simulink model "Battery_16EV_Cascaded_ACBus"  (R2026a)
settings: Solver=ode23t  StopTime=2
PreLoadFcn:
  | load('battery_pack_parameters.mat')
values from neighbouring files (symbols this model uses):
  branchSOH = [0.8 0.85 0.9 0.95 0.82 0.87 0.92 0.97 0.78 0.88 0.93 1 ... (16 elements, 1x16)]    [battery_pack_parameters.mat]
  packs =     [battery_bms_parameters.mat]    (also in battery_pack_parameters.mat)
libraries: fl_lib x145, nesl_utility x128, ee_lib x80, simulink x17, batteryecm_lib x16
(part 3 of 16)

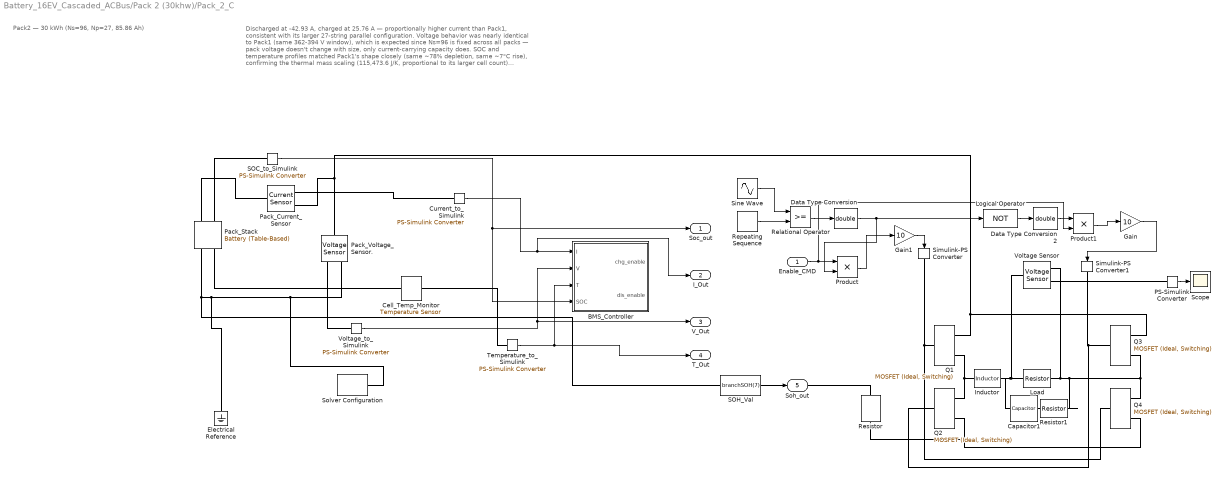
== system Battery_16EV_Cascaded_ACBus/Pack 2 (30khw)/Pack_2_C ==
  note: Discharged at -42.93 A, charged at 25.76 A — proportionally higher current than Pack1, consistent with its larger 27-string parallel configuration. Voltage behavior was nearly identical to Pack1 (same 362-394 V window), which is expected since Ns=96 is fixed across all packs — pack voltage doesn't change with size, only current-carrying capacity does. SOC and temperature profiles matched Pack1's shape closely (same ~78% depletion, same ~7°C rise), confirming the thermal mass scaling (115,473.6 J/K, proportional to its larger cell count) correctly absorbed the proportionally larger heat generation.
  note: Pack2 — 30 kWh (Ns=96, Np=27, 85.86 Ah)
  Enable_CMD : Inport
  BMS_Controller : MATLAB Function  TreatAsAtomicUnit=on
  Capacitor1 : ee_lib/Passive/Capacitor  cap_option=ee.enum.passive.capacitor.capOption.const  c=10e-6 F  Cvec=[1e-05, 1e-06] F  Vvec=[0, 10] V  CV_table_symmetry=ee.enum.passive.capacitor.tableSymmetry.yes  f_vec=[1, 10] kHz  DFext_vec=[.8, 1.2]  enable_C_tol=ee.enum.toleranceApplication.none  averaging_period=0 s  C_tol=5  tol_distribution=ee.enum.toleranceDistribution.uniform  nSigma=4  r=0 Ohm  g=0 1/Ohm  enable_operating_limits=ee.enum.enable.no  operating_limit_action=ee.enum.passive.reportOpLim.warn  max_working_voltage_range=[-25, 25] V  power_rating=1 W  maxTemperature=85 degC  thermalEnable=false  thermalMass=1 J/K  i_specify=off  i_priority=None  i=0 A  i_nominal_specify=off  i_nominal_value=1  i_nominal_unit=A  v_specify=off  v_priority=None  v=0 V  v_nominal_specify=off  v_nominal_value=1  v_nominal_unit=V  vc_specify=off  vc_priority=High  vc=0 V  vc_nominal_specify=off  vc_nominal_value=1  vc_nominal_unit=V  T_specify=off  T_priority=None  T=298.15 K  T_nominal_specify=off  T_nominal_value=1  T_nominal_unit=K
  Cell_Temp_Monitor : fl_lib/Thermal/Thermal Sensors/Temperature Sensor  temperature_measure=foundation.enum.MeasurementReference.absolute
  Current_to_Simulink : nesl_utility/PS-Simulink Converter  PhysicalDomain=network_engine_domain  SubClassName=ps_output  LeftPortType=input  RightPortType=output  PseudoPeriodic=off  Frequencies=[]  VectorFormat=inherit  Unit=inherit  AffineConversion=off
  Data Type Conversion : DataTypeConversion  OutDataTypeStr=double  SaturateOnIntegerOverflow=off  RndMeth=Floor
  Data Type Conversion2 : DataTypeConversion  OutDataTypeStr=double  SaturateOnIntegerOverflow=off  RndMeth=Floor
  Electrical Reference : fl_lib/Electrical/Electrical Elements/Electrical Reference
  Gain : Gain  Gain=10
  Gain1 : Gain  Gain=10
  Inductor : fl_lib/Electrical/Electrical Elements/Inductor  l=2e-3 H  r=0 Ohm  g=1e-9 1/Ohm  i_specify=off  i_priority=None  i=0 A  i_nominal_specify=off  i_nominal_value=1  i_nominal_unit=A  v_specify=off  v_priority=None  v=0 V  v_nominal_specify=off  v_nominal_value=1  v_nominal_unit=V  i_L_specify=off  i_L_priority=High  i_L=0 A  i_L_nominal_specify=off  i_L_nominal_value=1  i_L_nominal_unit=A
  Load : fl_lib/Electrical/Electrical Elements/Resistor  R=10 Ohm  i_specify=off  i_priority=None  i=0 A  i_nominal_specify=off  i_nominal_value=1  i_nominal_unit=A  v_specify=off  v_priority=None  v=0 V  v_nominal_specify=off  v_nominal_value=1  v_nominal_unit=V
  Logical Operator : Logic  Operator=NOT  AllPortsSameDT=off  OutDataTypeStr=boolean
  PS-Simulink Converter : nesl_utility/PS-Simulink Converter  PhysicalDomain=network_engine_domain  SubClassName=ps_output  LeftPortType=input  RightPortType=output  PseudoPeriodic=off  Frequencies=[]  VectorFormat=inherit  Unit=inherit  AffineConversion=off
  Pack_Current_Sensor : fl_lib/Electrical/Electrical Sensors/Current Sensor
  Pack_Stack : batteryecm_lib/Battery (Table-Based)  PartSpecification="{\"CollectionId\":\"MW.SimscapeBatteryShared\",\"CollectionVersion\":\"1.0.0\",\"DatasetId\":\"Panasonic|NCR18650BD|simscape.battery.batteryTableBased\",\"DisplayName\":\"Panasonic:NCR18650BD\"}"  SOC_vec=packs(2).SOC  T_dependence=simscape.enum.tablebattery.temperature_dependence.no  prm_dir=simscape.enum.tablebattery.prm_dir.noCurrentDirectionality  T_vec=[-10 0 25 40 60] % Datasheet derived degC  V0_mat=[2.90003 2.90003 2.90003 2.90003 2.90003;2.94341 2.94341 2.94341 2.94341 2.94341;2.98679 2.98679 2.98679 2.98679 2.98679;3.04987 3.04987 3.04987 3.04987 3.04987;3.09433 3.09433 3.09433 3.09433 3.09433;3.12791 3.12791 3.12791 3.12791 3.12791;3.16031 3.16031 3.16031 3.16031 3.16031;3.20369 3.20369 3.20369 3.20369 3.20369;3.23862 3.23862 3.23862 3.23862 3.23862;3.26689 3.26689 3.26689 3.26689 3.26689;3.29115 3.29115 3.29115 3.29115 3.29115;3.31383 3.31383 3.31383 3.31383 3.31383;3.33202 3.33202 3.33202 3.33202 3.33202;3.35112 3.35112 3.35112 3.35112 3.35112;3.36833 3.36833 3.36833 3.36833 3.36833;3.38413 3.38413 3.38413 3.38413 3.38413;3.39973 3.39973 3.39973 3.39973 3.39973;3.41137 3.41137 3.41137 3.41137 3.41137;3.42149 3.42149 3.42149 3.42149 3.42149;3.43136 3.43136 3.43136 3.43136 3.43136;3.44073 3.44073 3.44073 3.44073 3.44073;3.45027 3.45027 3.45027 3.45027 3.45027;3.46068 3.46068 3.46068 3.46068 3.46068;3.47113 3.47113 3.47113 3.47113 3.47113;3.47814 3.47814 3.47814 3.47814 3.47814;3.48494 3.48494 3.48494 3.48494 3.48494;3.49199 3.49199 3.49199 3.49199 3.49199;3.49905 3.49905 3.49905 3.49905 3.49905;3.50562 3.50562 3.50562 3.50562 3.50562;3.51187 3.51187 3.51187 3.51187 3.51187;3.51861 3.51861 3.51861 3.51861 3.51861;3.52535 3.52535 3.52535 3.52535 3.52535;3.53209 3.53209 3.53209 3.53209 3.53209;3.53818 3.53818 3.53818 3.53818 3.53818;3.54353 3.54353 3.54353 3.54353 3.54353;3.54849 3.54849 3.54849 3.54849 3.54849;3.55353 3.55353 3.55353 3.55353 3.55353;3.55855 3.55855 3.55855 3.55855 3.55855;3.56357 3.56357 3.56357 3.56357 3.56357;3.56831 3.56831 3.56831 3.56831 3.56831;3.57308 3.57308 3.57308 3.57308 3.57308;3.57787 3.57787 3.57787 3.57787 3.57787;3.58264 3.58264 3.58264 3.58264 3.58264;3.58755 3.58755 3.58755 3.58755 3.58755;3.5925 3.5925 3.5925 3.5925 3.5925;3.5985 3.5985 3.5985 3.5985 3.5985;3.60496 3.60496 3.60496 3.60496 3.60496;3.61149 3.61149 3.61149 3.61149 3.61149;3.61805 3.61805 3.61805 3.61805 3.61805;3.6246 3.6246 3.6246 3.6246 3.6246;3.63116 3.63116 3.63116 3.63116 3.63116;3.63855 3.63855 3.63855 3.63855 3.63855;3.64609 3.64609 3.64609 3.64609 3.64609;3.65336 3.65336 3.65336 3.65336 3.65336;3.66064 3.66064 3.66064 3.66064 3.66064;3.66791 3.66791 3.66791 3.66791 3.66791;3.67613 3.67613 3.67613 3.67613 3.67613;3.68522 3.68522 3.68522 3.68522 3.68522;3.69443 3.69443 3.69443 3.69443 3.69443;3.70367 3.70367 3.70367 3.70367 3.70367;3.713 3.713 3.713 3.713 3.713;3.72241 3.72241 3.72241 3.72241 3.72241;3.73154 3.73154 3.73154 3.73154 3.73154;3.74037 3.74037 3.74037 3.74037 3.74037;3.7492 3.7492 3.7492 3.7492 3.7492;3.75786 3.75786 3.75786 3.75786 3.75786;3.76617 3.76617 3.76617 3.76617 3.76617;3.77556 3.77556 3.77556 3.77556 3.77556;3.78485 3.78485 3.78485 3.78485 3.78485;3.79413 3.79413 3.79413 3.79413 3.79413;3.8034 3.8034 3.8034 3.8034 3.8034;3.81149 3.81149 3.81149 3.81149 3.81149;3.81977 3.81977 3.81977 3.81977 3.81977;3.82804 3.82804 3.82804 3.82804 3.82804;3.83631 3.83631 3.83631 3.83631 3.83631;3.84472 3.84472 3.84472 3.84472 3.84472;3.85317 3.85317 3.85317 3.85317 3.85317;3.86155 3.86155 3.86155 3.86155 3.86155;3.86993 3.86993 3.86993 3.86993 3.86993;3.87831 3.87831 3.87831 3.87831 3.87831;3.88686 3.88686 3.88686 3.88686 3.88686;3.89534 3.89534 3.89534 3.89534 3.89534;3.90461 3.90461 3.90461 3.90461 3.90461;3.91454 3.91454 3.91454 3.91454 3.91454;3.92565 3.92565 3.92565 3.92565 3.92565;3.93721 3.93721 3.93721 3.93721 3.93721;3.94924 3.94924 3.94924 3.94924 3.94924;3.96155 3.96155 3.96155 3.96155 3.96155;3.97383 3.97383 3.97383 3.97383 3.97383;3.98598 3.98598 3.98598 3.98598 3.98598;3.99856 3.99856 3.99856 3.99856 3.99856;4.01117 4.01117 4.01117 4.01117 4.01117;4.02361 4.02361 4.02361 4.02361 4.02361;4.03609 4.03609 4.03609 4.03609 4.03609;4.04694 4.04694 4.04694 4.04694 4.04694;4.05695 4.05695 4.05695 4.05695 4.05695;4.06641 4.06641 4.06641 4.06641 4.06641;4.07551 4.07551 4.07551 4.07551 4.07551;4.08514 4.08514 4.08514 4.08514 4.08514;4.09447 4.09447 4.09447 4.09447 4.09447;4.10453 4.10453 4.10453 4.10453 4.10453] % Datasheet derived V  V0_vec=packs(2).V0 V  V_range=[packs(2).V_min, max(packs(2).V0) + 17.3903] V  R0_mat=[0.54124 0.47218 0.1741 0.16472 0.13072;0.60048 0.51942 0.15823 0.09801 0.03241;0.57827 0.49613 0.14313 0.06257 0.00499;0.55606 0.47283 0.13285 0.0492 0.00058;0.53384 0.44953 0.12044 0.03857 0.00058;0.51163 0.42624 0.10641 0.0337 0.00058;0.48942 0.40294 0.09605 0.03258 0.00058;0.46721 0.37965 0.09162 0.03508 0.0103;0.44499 0.35635 0.08758 0.0376 0.01722;0.42278 0.33305 0.08349 0.04115 0.02235;0.40057 0.30976 0.08021 0.04338 0.0273;0.37836 0.28646 0.07738 0.04509 0.03173;0.35615 0.26317 0.07487 0.04551 0.03469;0.33393 0.24021 0.07338 0.04781 0.03783;0.31172 0.21801 0.07189 0.04948 0.04012;0.28951 0.203 0.07117 0.05069 0.04195;0.26873 0.19013 0.0704 0.05182 0.04371;0.24946 0.17834 0.06898 0.05166 0.04417;0.23189 0.16793 0.06755 0.05143 0.04397;0.21926 0.15878 0.06631 0.0513 0.04362;0.2084 0.15119 0.06509 0.05101 0.04311;0.19882 0.14534 0.06388 0.05077 0.04265;0.19282 0.14029 0.06326 0.05091 0.04272;0.18782 0.13679 0.06281 0.05124 0.04325;0.18252 0.13215 0.06182 0.05043 0.04264;0.17725 0.12766 0.06095 0.04955 0.04196;0.173 0.125 0.06025 0.04876 0.04137;0.16875 0.12234 0.05955 0.04802 0.04078;0.16459 0.11952 0.05877 0.04782 0.04033;0.16124 0.11704 0.05807 0.04752 0.03993;0.15805 0.11494 0.05761 0.04737 0.03969;0.15486 0.11285 0.05714 0.04723 0.03945;0.15212 0.11075 0.05668 0.04709 0.03921;0.15022 0.10906 0.05611 0.04673 0.03878;0.14807 0.10773 0.05546 0.04612 0.03867;0.14579 0.10628 0.0549 0.04546 0.03843;0.14353 0.10484 0.05439 0.04485 0.03821;0.14127 0.10351 0.05388 0.04423 0.03799;0.13957 0.10228 0.05337 0.04361 0.03777;0.13785 0.10097 0.0528 0.0429 0.03746;0.13614 0.09966 0.05223 0.0422 0.0367;0.13443 0.09836 0.05165 0.04151 0.03572;0.13272 0.09711 0.05106 0.04111 0.03474;0.13096 0.09591 0.05046 0.04079 0.03381;0.12918 0.09471 0.04986 0.04049 0.03288;0.12775 0.09387 0.04945 0.04053 0.03231;0.12648 0.09317 0.04913 0.04073 0.03189;0.12522 0.09249 0.04883 0.04095 0.03151;0.12398 0.09181 0.04854 0.04066 0.03136;0.12296 0.09112 0.04826 0.04006 0.03121;0.12207 0.09044 0.04797 0.03947 0.03106;0.12147 0.09003 0.04782 0.03916 0.03119;0.12091 0.08967 0.04765 0.03889 0.03136;0.12027 0.08886 0.0473 0.03854 0.03145;0.11955 0.08797 0.04695 0.03818 0.03154;0.11836 0.08708 0.04661 0.03764 0.03136;0.11749 0.08651 0.04638 0.03733 0.03126;0.1169 0.08628 0.0463 0.03731 0.03144;0.11636 0.0866 0.04625 0.03733 0.03167;0.11679 0.08693 0.04621 0.03736 0.0319;0.11639 0.08729 0.04624 0.03741 0.03216;0.11602 0.08748 0.04628 0.0375 0.03245;0.11556 0.08747 0.04628 0.03749 0.03262;0.115 0.08737 0.04623 0.03738 0.03268;0.11444 0.08726 0.04617 0.03728 0.03275;0.11413 0.08683 0.04599 0.03714 0.03276;0.11369 0.08629 0.04573 0.03712 0.03265;0.11362 0.0861 0.0457 0.03746 0.03289;0.11351 0.08597 0.04568 0.03777 0.03289;0.1134 0.08596 0.04565 0.03807 0.03285;0.11329 0.08593 0.04563 0.03837 0.0328;0.11297 0.08552 0.04535 0.03804 0.03236;0.1131 0.0855 0.0451 0.03769 0.03198;0.11323 0.08564 0.04486 0.03733 0.0316;0.11336 0.08578 0.04461 0.03698 0.03122;0.11354 0.08596 0.04446 0.03667 0.03091;0.11376 0.08614 0.04435 0.03629 0.0306;0.11421 0.08628 0.04423 0.03577 0.03027;0.11467 0.08641 0.04411 0.03525 0.02995;0.11513 0.08655 0.044 0.03473 0.02961;0.11565 0.08679 0.04372 0.03426 0.02933;0.11614 0.08704 0.04339 0.03378 0.02903;0.11689 0.08756 0.04323 0.03353 0.02899;0.11825 0.08829 0.0432 0.03328 0.02916;0.12033 0.08941 0.04344 0.03342 0.02973;0.12256 0.09067 0.04374 0.03371 0.0301;0.12495 0.09191 0.0441 0.03415 0.02981;0.12743 0.09323 0.04452 0.03468 0.0296;0.13108 0.09454 0.04494 0.03488 0.02939;0.13509 0.09581 0.0454 0.03488 0.02914;0.13924 0.09835 0.04594 0.03502 0.02907;0.14357 0.1012 0.0463 0.03517 0.02937;0.14857 0.10399 0.04649 0.03528 0.02963;0.15358 0.10679 0.04668 0.03541 0.02989;0.15894 0.10894 0.04629 0.035 0.02961;0.16451 0.11073 0.04541 0.03434 0.02892;0.17255 0.11235 0.04438 0.03375 0.02804;0.17994 0.11383 0.04326 0.03305 0.02704;0.18615 0.11422 0.04154 0.03252 0.02601;0.19123 0.11362 0.03869 0.03189 0.02484;0.17773 0.09538 0.03326 0.0315 0.0239] % Datasheet derived Ohm  R0_vec=packs(2).R0 Ohm  R0_dis_mat=[.0117, .0085, .009; .011, .0085, .009; .0114, .0087, .0092; .0107, .0082, .0088; .0107, .0083, .0091; .0113, .0085, .0089; .0116, .0085, .0089] % Parameter not set Ohm  R0_dis_vec=[.0085, .0085, .0087, .0082, .0083, .0085, .0085] % Parameter not set Ohm  R0_ch_mat=[.0117, .0085, .009; .011, .0085, .009; .0114, .0087, .0092; .0107, .0082, .0088; .0107, .0083, .0091; .0113, .0085, .0089; .0116, .0085, .0089] % Parameter not set Ohm  R0_ch_vec=[.0085, .0085, .0087, .0082, .0083, .0085, .0085] % Parameter not set Ohm  AH=packs(2).capacity_Ah * branchSOH(7) hr*A  prm_leak=simscape.enum.tablebattery.prm_leak.disabled  Rleak_vec=[8000, 7000, 6000] % Parameter not set Ohm  Rleak=7e3 % Parameter not set Ohm  extrapolation_option=simscape.enum.extrapolation.nearest  SOC_port=simscape.enum.tablebattery.enable.yes  prm_dyn=simscape.enum.tablebattery.prm_dyn.off  R1_mat=[.0109, .0029, .0013; .0069, .0024, .0012; .0047, .0026, .0013; .0034, .0016, .001; .0033, .0023, .0014; .0033, .0018, .0011; .0028, .0017, .0011] % Parameter not set Ohm  R1_vec=[.0029, .0024, .0026, .0016, .0023, .0018, .0017] % Parameter not set Ohm  tau1_mat=[20, 36, 39; 31, 45, 39; 109, 105, 61; 36, 29, 26; 59, 77, 67; 40, 33, 29; 25, 39, 33] % Parameter not set s  tau1_vec=[36, 45, 105, 29, 77, 33, 39] % Parameter not set s  R2_mat=[.0109, .0029, .0013; .0069, .0024, .0012; .0047, .0026, .0013; .0034, .0016, .001; .0033, .0023, .0014; .0033, .0018, .0011; .0028, .0017, .0011] % Parameter not set Ohm  R2_vec=[.0029, .0024, .0026, .0016, .0023, .0018, .0017] % Parameter not set Ohm  tau2_mat=[20, 36, 39; 31, 45, 39; 109, 105, 61; 36, 29, 26; 59, 77, 67; 40, 33, 29; 25, 39, 33] % Parameter not set s  tau2_vec=[36, 45, 105, 29, 77, 33, 39] % Parameter not set s  R3_mat=[.0109, .0029, .0013; .0069, .0024, .0012; .0047, .0026, .0013; .0034, .0016, .001; .0033, .0023, .0014; .0033, .0018, .0011; .0028, .0017, .0011] % Parameter not set Ohm  R3_vec=[.0029, .0024, .0026, .0016, .0023, .0018, .0017] % Parameter not set Ohm  tau3_mat=[20, 36, 39; 31, 45, 39; 109, 105, 61; 36, 29, 26; 59, 77, 67; 40, 33, 29; 25, 39, 33] % Parameter not set s  tau3_vec=[36, 45, 105, 29, 77, 33, 39] % Parameter not set s  R4_mat=[.0109, .0029, .0013; .0069, .0024, .0012; .0047, .0026, .0013; .0034, .0016, .001; .0033, .0023, .0014; .0033, .0018, .0011; .0028, .0017, .0011] % Parameter not set Ohm  R4_vec=[.0029, .0024, .0026, .0016, .0023, .0018, .0017] % Parameter not set Ohm  tau4_mat=[20, 36, 39; 31, 45, 39; 109, 105, 61; 36, 29, 26; 59, 77, 67; 40, 33, 29; 25, 39, 33] % Parameter not set s  tau4_vec=[36, 45, 105, 29, 77, 33, 39] % Parameter not set s  R5_mat=[.0109, .0029, .0013; .0069, .0024, .0012; .0047, .0026, .0013; .0034, .0016, .001; .0033, .0023, .0014; .0033, .0018, .0011; .0028, .0017, .0011] % Parameter not set Ohm  R5_vec=[.0029, .0024, .0026, .0016, .0023, .0018, .0017] % Parameter not set Ohm  tau5_mat=[20, 36, 39; 31, 45, 39; 109, 105, 61; 36, 29, 26; 59, 77, 67; 40, 33, 29; 25, 39, 33] % Parameter not set s  tau5_vec=[36, 45, 105, 29, 77, 33, 39] % Parameter not set s  prm_fade=simscape.enum.tablebattery.prm_fade.tableN  N0=100 % Parameter not set  dV0=0 % Parameter not set  dR0=0 % Parameter not set  dAH=0 % Parameter not set  dRleak=0 % Parameter not set  dR1=0 % Parameter not set  dR2=0 % Parameter not set  dR3=0 % Parameter not set  dR4=0 % Parameter not set  dR5=0 % Parameter not set  N0vec=[0 5 9 13 17 21 25 29 33 37 41 45 49 53 57 61 65 69 73 77 81 85 89 93 97 101 105 109 113 117 121 125 129 133 137 141 145 149 153 157 161 165 169 173 177 181 185 189 193 197 201 205 209 213 217 221 225 229 233 237 241 245 249 253 257 261 265 269 273 277 281 285 289 293 297 301 305 309 313 317] % Datasheet derived  Tfadevec=[298.15, 323.15] % Parameter not set K  dV0vec=[0 -0.2107 -0.4072 -0.4916 -0.5781 -0.6646 -0.7487 -0.8154 -0.8801 -0.9454 -1.0127 -1.08 -1.1384 -1.1799 -1.2225 -1.2652 -1.3079 -1.3505 -1.3932 -1.4386 -1.4849 -1.5273 -1.567 -1.6067 -1.6464 -1.6889 -1.7346 -1.7803 -1.826 -1.8717 -1.9175 -1.9634 -2.0091 -2.0549 -2.1006 -2.1463 -2.1921 -2.2378 -2.2801 -2.3167 -2.3534 -2.39 -2.4267 -2.4633 -2.4999 -2.5366 -2.5732 -2.6098 -2.6449 -2.6793 -2.7137 -2.7482 -2.7826 -2.817 -2.8515 -2.8859 -2.9192 -2.9512 -2.9793 -3.0074 -3.0355 -3.0636 -3.0917 -3.1198 -3.1479 -3.1758 -3.2018 -3.2279 -3.254 -3.2801 -3.3062 -3.3323 -3.3605 -3.3912 -3.4219 -3.4526 -3.4833 -3.5141 -3.5449 -3.5756] % Datasheet derived  dR0vec=[0 0 0 0 0 0 0 0 0 0 0 0 0 0 0 0 0 0 0 0 0 0 0 0 0 0 0 0 0 0 0 0 0 0 0 0 0 0 0 0 0 0 0 0 0 0 0 0 0 0 0 0 0 0 0 0 0 0 0 0 0 0 0 0 0 0 0 0 0 0 0 0 0 0 0 0 0 0 0 0] % Parameter assumed  dAHvec=[0 -0.86 -1.713 -2.082 -2.451 -2.819 -3.188 -3.489 -3.781 -4.073 -4.365 -4.657 -4.91 -5.085 -5.26 -5.435 -5.61 -5.785 -5.96 -6.135 -6.31 -6.47 -6.62 -6.771 -6.921 -7.071 -7.221 -7.371 -7.522 -7.672 -7.822 -7.973 -8.124 -8.275 -8.426 -8.577 -8.728 -8.879 -9.018 -9.137 -9.256 -9.376 -9.495 -9.614 -9.734 -9.853 -9.972 -10.091 -10.206 -10.318 -10.431 -10.543 -10.655 -10.768 -10.88 -10.992 -11.105 -11.213 -11.308 -11.403 -11.498 -11.593 -11.687 -11.782 -11.877 -11.972 -12.059 -12.146 -12.233 -12.321 -12.408 -12.495 -12.589 -12.692 -12.794 -12.897 -12.999 -13.102 -13.205 -13.307] % Datasheet derived  dRleakvec=[0, 0, 0, 0] % Parameter not set  dR1vec=[0, 0, 0, 0] % Parameter not set  dR2vec=[0, 0, 0, 0] % Parameter not set  dR3vec=[0, 0, 0, 0] % Parameter not set  dR4vec=[0, 0, 0, 0] % Parameter not set  dR5vec=[0, 0, 0, 0] % Parameter not set  dV0mat=[0, 0; 0, 0; 0, 0; 0, 0] % Parameter not set  dR0mat=[0, 0; 0, 0; 0, 0; 0, 0] % Parameter not set  dAHmat=[0, 0; 0, 0; 0, 0; 0, 0] % Parameter not set  dRleakmat=[0, 0; 0, 0; 0, 0; 0, 0] % Parameter not set  dR1mat=[0, 0; 0, 0; 0, 0; 0, 0] % Parameter not set  dR2mat=[0, 0; 0, 0; 0, 0; 0, 0] % Parameter not set  dR3mat=[0, 0; 0, 0; 0, 0; 0, 0] % Parameter not set  dR4mat=[0, 0; 0, 0; 0, 0; 0, 0] % Parameter not set  dR5mat=[0, 0; 0, 0; 0, 0; 0, 0] % Parameter not set  prm_age_modeling=simscape.enum.tablebattery.prm_age_modeling.equation  storage_dt_age_vec=[0] % Parameter not set d  storage_T_age_vec=[273] % Parameter not set K  prm_age_OCV=simscape.enum.tablebattery.prm_age_OCV.OCV  OCV_age=0.9 % Parameter not set  SOC_age=0.6 % Parameter not set  prm_age_resistance=simscape.enum.tablebattery.prm_age.disabled  OCV_scaling_age_resistance=2.2134e6 % Parameter not set  OCV_offset_age_resistance=1.632e6 % Parameter not set  temp_exp_age_resistance=0.515833569 % Parameter not set V  t_exp_age_resistance=0.75 % Parameter not set  T_age_vec_resistance=[273.15, 298.15, 323.15] % Parameter not set K  dt_age_vec_resistance=[0, 90, 180, 270] % Parameter not set d  dR0_age_vec=[0, 0, 0] % Parameter not set  t_meas_dR0_age=100 % Parameter not set d  dR0_age_mat=[0, 0, 0; 0, 0, 0; 0, 0, 0; 0, 0, 0] % Parameter not set  prm_age_capacity=simscape.enum.tablebattery.prm_age.disabled  OCV_scaling_age_capacity=1.5097e07 % Parameter not set  OCV_offset_age_capacity=8.3625e06 % Parameter not set  temp_exp_age_capacity=0.6011 % Parameter not set V  t_exp_age_capacity=0.75 % Parameter not set  T_age_vec_capacity=[273.15, 298.15, 323.15] % Parameter not set K  dt_age_vec_capacity=[0, 90, 180, 270] % Parameter not set d  dAH_age_vec=[0, 0, 0] % Parameter not set  t_meas_dAH_age=100 % Parameter not set d  dAH_age_mat=[0, 0, 0; 0, 0, 0; 0, 0, 0; 0, 0, 0] % Parameter not set  thermal_port=simscape.enum.thermaleffects.model  temperature=298.15 + (1 - branchSOH(7)) * 15 / (1 - 0.78) K  thermal_mass=packs(2).Ns * packs(2).Np * 44.55 J/K  i_specify=off  i_priority=None  i=0 A  i_nominal_specify=off  i_nominal_value=1  i_nominal_unit=A  v_specify=off  v_priority=None  v=0 V  v_nominal_specify=off  v_nominal_value=1  v_nominal_unit=V  stateOfCharge_specify=on  stateOfCharge_priority=High  stateOfCharge=1  stateOfCharge_nominal_specify=off  stateOfCharge_nominal_value=1.00  stateOfCharge_nominal_unit=1  num_cycles_specify=off  num_cycles_priority=High  num_cycles=0  num_cycles_nominal_specify=off  num_cycles_nominal_value=1  num_cycles_nominal_unit=1  cell_temperature_specify=on  cell_temperature_priority=High  cell_temperature=298.15 + (1 - branchSOH(7)) * 15 / (1 - 0.78) K  cell_temperature_nominal_specify=off  cell_temperature_nominal_value=1  cell_temperature_nominal_unit=K
      settings: AttributesFormatString=Panasonic:NCR18650BD
      settings: LibrarySourceBlock=|
      | batt_lib/Cells/Battery
      | (Table-Based)
  Pack_Voltage_Sensor. : fl_lib/Electrical/Electrical Sensors/Voltage Sensor
  Product : Product
  Product1 : Product
  Q{1..4} (4 alike) : ee_lib/Semiconductors & Converters/MOSFET (Ideal, Switching)  port_option=ee.enum.controlport.ps  Rds=0.01 Ohm  Goff=1e-6 1/Ohm  Vth=2 V  diode_param=ee.enum.semiconductors.protectionDiode.nodynamics  diode_Vf=0.8 V  diode_Ron=0.001 Ohm  diode_Goff=1e-5 1/Ohm  diode_C=50e-9 F  diode_iRM=-235 A  diode_iF=300 A  diode_idot=-50 A/us  diode_trr_param=ee.enum.converters.diodeReverseParam.trr_factor  diode_trr_factor=3  diode_trr=15 us  diode_Qrr=1500 s*uA  ids_specify=off  ids_priority=None  ids=0 A  ids_nominal_specify=off  ids_nominal_value=1  ids_nominal_unit=A  vds_specify=off  vds_priority=None  vds=0 V  vds_nominal_specify=off  vds_nominal_value=1  vds_nominal_unit=V  vgs_specify=off  vgs_priority=None  vgs=0 V  vgs_nominal_specify=off  vgs_nominal_value=1  vgs_nominal_unit=V  thermal_loss_option=ee.enum.converters.thermalLossOption.constantvalues  Von_data=[0, 1.8, 3.2, 6, 10, 16; 0, 2, 5.5, 9.5, 15, 25] V  Tj=[298.15, 448.15] K  Iout_data=[0, 20, 40, 60, 80, 100] A  tabulateWithVds=false  Eon_data=[0, 55.04, 124.57, 235.53, 362.12; 0, 71.25, 161.25, 304.88, 468.75] * 1e-6 J  Eoff_data=[0, 18, 30, 56.1, 76.5; 0, 22.5, 37.5, 70.13, 95.63] * 1e-6 J  Eon_data_3D=[zeros(2, 5, 3)] J  Eoff_data_3D=[zeros(2, 5, 3)] J  Tj_loss=[298.15, 448.15] K  Iout_data_loss=[0, 10, 20, 30, 40] A  Vds_loss=[0, 150, 300] V  Eon_scalar=22.86e-3 J  Eoff_scalar=17.14e-3 J  Voff=300 V  Iout_scalar=600 A  useCurrentFromPreviousCycle=false  useVoltageFromPreviousCycle=false  diodeModelType=ee.enum.converters.diodeModelType.pwl  diodeTableType=ee.enum.diode.tableType.IfMat  diode_ReverseIVType=ee.enum.diode.diodeReverseIV.constant  diode_IfMat=[.07, .12, .19, 1.75, 4.24, 7.32, 11.2; .16, .3, .72, 2.14, 4.02, 6.35, 9.12] A  diode_VfMat=[.9, 1.15, 1.25, 1.5, 1.75, 2.17, 2.6, 2.85; .58, .68, .75, 1.1, 1.38, 1.77, 2.27, 2.7] V  diode_TjVec=[25, 125] degC  diode_VfVec=[.5, .7, .9, 1.3, 1.7, 2.1, 2.5] V  diode_IfVec=[.1, .2, .5, 1, 2, 4, 7, 10] A  diode_IrMat=[1e-06, 2e-06, 5e-06, 1e-05, 2.5e-05, 5e-05, .0001; 2e-06, 5e-06, 1e-05, 4e-05, 8e-05, .0002, .0005] A  diode_VrMat=[10, 100, 200, 250, 300, 325, 350; 10, 70, 160, 220, 270, 300, 320] V  diode_VrVec=[10, 20, 40, 50, 70, 80, 100] V  diode_IrVec=[1e-06, 2e-06, 5e-06, 1e-05, 2e-05, 5e-05, .0001] A  diode_Vr=-600 V  diode_Ls=150 nH  diode_Erec=0.03 J  diode_rec_loss_model=ee.enum.diode.reverseRecoveryModel.fixed  diode_ErecVal=0 J  diode_scaleWithIandV=true  diode_ErecMat=zeros(2, 3) J  diodeErecMat3D=zeros(2, 3, 2) J  diode_TjrecVec=[298.15, 398.15] K  diode_IfrecVec=[.1, 1, 10] A  diodeVrecVec=[0, 100] V  diode_IrecVal=10 A  diode_VrecVal=10 V  diode_tFilter=1 / 1000 / 100 s  separateThermalPortForDiode=false  thermal_network_parameterization=ee.enum.thermalNetworkTopology.external  Rth=[.03, .2] K/W  Rth_Cauer=[.03, .1, .2] K/W  Rth_Foster=[.08, .14, .22, .16] K/W  thermal_mass_parameterization=ee.enum.thermalNetwork.timeconstant  thermal_mass=[3, 25] J/K  thermal_mass_Cauer=[3, 10, 25] J/K  thermal_mass_Foster=[.001, .005, .05, .5] J/K  thermal_time_constant=[.1, 5] s  thermal_time_constant_Cauer=[.1, 1, 5] s  thermal_time_constant_Foster=[7e-05, .0007, .01, .08] s  thermal_mass_initial_temperatures=[25, 25] degC  thermal_mass_initial_temperatures_Cauer=[25, 25, 25] degC  junction_thermal_mass=0.1 J/K  Tvec_initial_Foster=[25, 25, 25, 25] degC  RthDiode=[.03, .2] K/W  RthCauerDiode=[.03, .1, .2] K/W  RthFosterDiode=[.03, .2] K/W  thermalMassDiode=[3, 25] J/K  thermalMassCauerDiode=[3, 10, 25] J/K  thermalMassFosterDiode=[33, 50] J/K  thermalTauDiode=[.1, 5] s  thermalTauCauerDiode=[.1, 1, 5] s  thermalTauFosterDiode=[1, 10] s  thermalMassInitTempDiode=[25, 25] degC  thermalMassInitTempCauerDiode=[25, 25, 25] degC  junctionthermalMassDiode=0.1 J/K  TVecInitialFosterDiode=[25, 25, 25, 25] degC  no_thermal_network=0  mosfet_junction_temperature_specify=off  mosfet_junction_temperature_priority=None  mosfet_junction_temperature=25 degC  mosfet_junction_temperature_nominal_specify=off  mosfet_junction_temperature_nominal_value=1  mosfet_junction_temperature_nominal_unit=degC  diode_junction_temperature_specify=off  diode_junction_temperature_priority=None  diode_junction_temperature=25 degC  diode_junction_temperature_nominal_specify=off  diode_junction_temperature_nominal_value=1  diode_junction_temperature_nominal_unit=degC  Qj_specify=off  Qj_priority=None  Qj=0 W  Qj_nominal_specify=off  Qj_nominal_value=1  Qj_nominal_unit=W  accumulatedSwitchingLosses_specify=off  accumulatedSwitchingLosses_priority=None  accumulatedSwitchingLosses=0 J
  Relational Operator : RelationalOperator  OutDataTypeStr=boolean  RndMeth=Simplest  InputSameDT=off
  Repeating Sequence : simulink/Sources/Repeating Sequence  rep_seq_t=[0, (1/20000), (1/10000)]  rep_seq_y=[-1,1,-1]
  Resistor : fl_lib/Electrical/Electrical Elements/Resistor  R=1 Ohm  i_specify=off  i_priority=None  i=0 A  i_nominal_specify=off  i_nominal_value=1  i_nominal_unit=A  v_specify=off  v_priority=None  v=0 V  v_nominal_specify=off  v_nominal_value=1  v_nominal_unit=V
  Resistor1 : fl_lib/Electrical/Electrical Elements/Resistor  R=1 Ohm  i_specify=off  i_priority=None  i=0 A  i_nominal_specify=off  i_nominal_value=1  i_nominal_unit=A  v_specify=off  v_priority=None  v=0 V  v_nominal_specify=off  v_nominal_value=1  v_nominal_unit=V
  SOC_to_Simulink : nesl_utility/PS-Simulink Converter  PhysicalDomain=network_engine_domain  SubClassName=ps_output  LeftPortType=input  RightPortType=output  PseudoPeriodic=off  Frequencies=[]  VectorFormat=inherit  Unit=inherit  AffineConversion=off
  SOH_Val : Constant  Value=branchSOH(7)
  Scope : Scope
      settings: ActiveDisplayYMinimum=15.720292471792343  ActiveDisplayYMaximum=24.108244369256735  DataLoggingVariableName=ScopeData21
  Simulink-PS Converter : nesl_utility/Simulink-PS Converter  PhysicalDomain=network_engine_domain  SubClassName=ps_input  LeftPortType=input  RightPortType=output  PseudoPeriodic=off  Frequencies=[]  NoiseDistribution=none  NoiseParameters=[]  Unit=1  AffineConversion=off  FilteringAndDerivatives=zero  SimscapeFilterOrder=1  InputFilterTimeConstant=0.001  UdotUserProvided=0
  Simulink-PS Converter1 : nesl_utility/Simulink-PS Converter  PhysicalDomain=network_engine_domain  SubClassName=ps_input  LeftPortType=input  RightPortType=output  PseudoPeriodic=off  Frequencies=[]  NoiseDistribution=none  NoiseParameters=[]  Unit=1  AffineConversion=off  FilteringAndDerivatives=zero  SimscapeFilterOrder=1  InputFilterTimeConstant=0.001  UdotUserProvided=0
  Sine Wave : Sin  Amplitude=0.9  Frequency=2*pi*50  SampleTime=0
  Solver Configuration : nesl_utility/Solver Configuration  PhysicalDomain=network_engine_domain  SubClassName=solver  LeftPortType=input  RightPortType=generic  Tones=[]  Harmonics=[]  SimulateNoise=off  Profile=off  UseLocalSampling=off  EnableSwitchedLinearOptims=on  FrequencyDomain=off  UseCCode=off  RelTol=0.001  AbsTol=0.001  MinStep=1e-09  ToWorkspace=off  RevertToSquareIcSolve=off  NumHomotopyIterations=100  PhasorMode=off  PhasorModeNumHarmonics=1  ConsistencySolver=NEWTON_XTOL_AFTER_FTOL  CanonicalOrdering=CANONICAL  OptimizeIntermediates=OPTIMIZED  IndexReductionMethod=DerivativeReplacement  DoDC=off  ResidualTolerance=1e-09  ConsistencyTolSource=GLOBAL  ConsistencyAbsTol=0.001  ConsistencyRelTol=0.001  ConsistencyTolFactor=0.001  UseLocalSolver=off  LocalSolverChoice=NE_BACKWARD_EULER_ADVANCER  ResolveIndetEquations=on  FunctionEvalNumThread=1  LocalSolverSampleTime=0.001  DoFixedCost=off  MaxNonlinIter=3  MaxModeIter=2  ComputeImpulses=off  ImpulseIterations=2  LinearAlgebra=auto  LinearAlgebraNumThread=0  EquationFormulation=NE_TIME_EF  DelaysMemoryBudget=1024  AutomaticFiltering=on  FilteringTimeConstant=0.001  PartitionStorageMethod=AS_NEEDED  PartitionMemoryBudget=1024  PartitionMethod=ROBUST  MultibodyUseLocalSolver=off  MultibodyLocalSolverChoice=ODE1  MultibodyLocalSolverSampleTime=0.001
  Temperature_to_Simulink : nesl_utility/PS-Simulink Converter  PhysicalDomain=network_engine_domain  SubClassName=ps_output  LeftPortType=input  RightPortType=output  PseudoPeriodic=off  Frequencies=[]  VectorFormat=inherit  Unit=inherit  AffineConversion=off
  Voltage Sensor : fl_lib/Electrical/Electrical Sensors/Voltage Sensor
  Voltage_to_Simulink : nesl_utility/PS-Simulink Converter  PhysicalDomain=network_engine_domain  SubClassName=ps_output  LeftPortType=input  RightPortType=output  PseudoPeriodic=off  Frequencies=[]  VectorFormat=inherit  Unit=inherit  AffineConversion=off
  Soc_out : Outport
  I_Out : Outport  Port=2
  V_Out : Outport  Port=3
  T_Out : Outport  Port=4
  Soh_out : Outport  Port=5
  wires:
  Current_to_Simulink/1 -> I_Out/1, BMS_Controller/1(I)
  Voltage_to_Simulink/1 -> V_Out/1, BMS_Controller/2(V)
  Temperature_to_Simulink/1 -> T_Out/1, BMS_Controller/3(T)
  SOC_to_Simulink/1 -> BMS_Controller/4(SOC), Soc_out/1
  Gain/1 -> Simulink-PS Converter1/1
  Sine Wave/1 -> Relational Operator/1
  Data Type Conversion/1 -> Product/2, Logical Operator/1
  Logical Operator/1 -> Data Type Conversion2/1
  Repeating Sequence/1 -> Relational Operator/2
  Gain1/1 -> Simulink-PS Converter/1
  Relational Operator/1 -> Data Type Conversion/1
  PS-Simulink Converter/1 -> Scope/1
  SOH_Val/1 -> Soh_out/1
  Enable_CMD/1 -> Product1/2, Product/1
  Product/1 -> Gain1/1
  Data Type Conversion2/1 -> Product1/1
  Product1/1 -> Gain/1
  connections:
  Pack_Stack/RConn1 -- Resistor/LConn1 -- Electrical Reference/LConn1 -- Pack_Voltage_Sensor./RConn2 -- Solver Configuration/RConn1
  Cell_Temp_Monitor/LConn1 -- Pack_Stack/RConn2
  Current_to_Simulink/LConn1 -- Pack_Current_Sensor/RConn1
  Pack_Voltage_Sensor./RConn1 -- Voltage_to_Simulink/LConn1
  Cell_Temp_Monitor/RConn1 -- Temperature_to_Simulink/LConn1
  SOC_to_Simulink/LConn1 -- Pack_Stack/LConn2
  Q3/RConn1 -- Pack_Current_Sensor/RConn2 -- Pack_Voltage_Sensor./LConn1 -- Q1/RConn1
  Q4/RConn2 -- Resistor/RConn1 -- Q2/RConn2
  Q4/RConn1 -- Q3/RConn2 -- Voltage Sensor/RConn2 -- Load/RConn1 -- Resistor1/RConn1
  Q2/RConn1 -- Q1/RConn2 -- Inductor/LConn1
  Q2/LConn1 -- Simulink-PS Converter1/RConn1 -- Q3/LConn1
  Voltage Sensor/LConn1 -- Load/LConn1 -- Inductor/RConn1 -- Capacitor1/LConn1
  Q4/LConn1 -- Q1/LConn1 -- Simulink-PS Converter/RConn1
  PS-Simulink Converter/LConn1 -- Voltage Sensor/RConn1
  Resistor1/LConn1 -- Capacitor1/RConn1
  Pack_Stack/LConn1 -- Pack_Current_Sensor/LConn1
